simulink model "HybridShip_ModelE"  (R2026a)
settings: Solver=ode3  StopTime=7200  FixedStep=0.01
undefined symbols (not defined in the file): ADAPTER_FORCE_MODE, ADAPTER_FORCE_P1_KW, ADAPTER_FORCE_P2_KW, AI_Pred_Source, AI_TPeak_Source, ASSUMED_AI_DataValid, ASSUMED_Bat_Eff_Charge, ASSUMED_Bat_Eff_Discharge, ASSUMED_C_bus, ASSUMED_Drive_TimeConstant, ASSUMED_EMS_FF_Gain, ASSUMED_EMS_FF_Max_kW, ASSUMED_EMS_Manual_Pgen_kW, ASSUMED_EMS_SOC_Gain, ASSUMED_EMS_SOC_Ref, ASSUMED_eta_dcdc, ASSUMED_eta_rect, ASSUMED_Gen_TimeConstant, ASSUMED_K_droop, ASSUMED_Pred_Bound_kW, ASSUMED_SOC_ChgDerate_Start, ASSUMED_SOC_DisDerate_Start, ASSUMED_SOC_max, ASSUMED_SOC_min, ASSUMED_SpeedPI_Ki, ASSUMED_SpeedPI_Kp, ASSUMED_TFF_SOC_AdvancePct, ASSUMED_TFF_SOC_Thresh, ASSUMED_TFF_TauMargin, ASSUMED_V_floor, Bat_C1_LUT_F, Bat_eta_coul, Bat_I_limit_surrogate_A, Bat_OCV_LUT_V, Bat_P_conv_bus_max_kW, Bat_Q_nom_Ah, Bat_R0_chg_mult, Bat_R0_LUT_ohm, Bat_R1_LUT_ohm, Bat_SOC_init, Bat_SOC_LUT_nodes, Bat_V_max_V, Bat_V_min_V, BSFC_Breakpoints_kW, BSFC_Table_gkWh, CCS_Vdc_Steady_Band, CCS_Vdc_Transient_Band, DG_BSFC_gkWh, DG_BSFC_P_kW, DG_C_start_kg, DG_P_min_kW, DG_P_rated_kW, DG_ramp_kW_per_s, DG_t_starting_s, DG_t_sync_s, DG_tau_s, ECMS_dt_ctrl_s, ECMS_Grid_dP_kW, ECMS_Idle_Fuel_kgph, ECMS_K_S ... (+93)
libraries: simulink x8
(part 2 of 3)

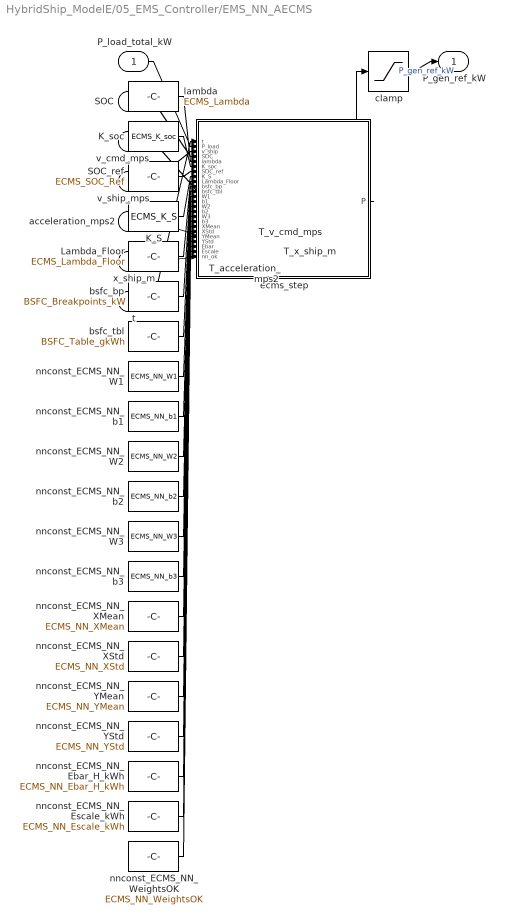
== system HybridShip_ModelE/05_EMS_Controller/EMS_NN_AECMS ==
  P_load_total_kW : Inport
  SOC : Inport  Port=2
  v_cmd_mps : Inport  Port=3
  v_ship_mps : Inport  Port=4
  acceleration_mps2 : Inport  Port=5
  x_ship_m : Inport  Port=6
  t : Inport  Port=7
  K_S : Constant  Value=ECMS_K_S
  K_soc : Constant  Value=ECMS_K_soc
  Lambda_Floor : Constant  Value=ECMS_Lambda_Floor
  SOC_ref : Constant  Value=ECMS_SOC_Ref
  T_acceleration_mps2 : Terminator
  T_v_cmd_mps : Terminator
  T_x_ship_m : Terminator
  bsfc_bp : Constant  Value=BSFC_Breakpoints_kW
  bsfc_tbl : Constant  Value=BSFC_Table_gkWh
  clamp : Saturate  UpperLimit=Gen_P_max  LowerLimit=0
  ecms_step : MATLAB Function  TreatAsAtomicUnit=on
  lambda : Constant  Value=ECMS_Lambda
  nnconst_ECMS_NN_Ebar_H_kWh : Constant  Value=ECMS_NN_Ebar_H_kWh
  nnconst_ECMS_NN_Escale_kWh : Constant  Value=ECMS_NN_Escale_kWh
  nnconst_ECMS_NN_W1 : Constant  Value=ECMS_NN_W1
  nnconst_ECMS_NN_W2 : Constant  Value=ECMS_NN_W2
  nnconst_ECMS_NN_W3 : Constant  Value=ECMS_NN_W3
  nnconst_ECMS_NN_WeightsOK : Constant  Value=ECMS_NN_WeightsOK
  nnconst_ECMS_NN_XMean : Constant  Value=ECMS_NN_XMean
  nnconst_ECMS_NN_XStd : Constant  Value=ECMS_NN_XStd
  nnconst_ECMS_NN_YMean : Constant  Value=ECMS_NN_YMean
  nnconst_ECMS_NN_YStd : Constant  Value=ECMS_NN_YStd
  nnconst_ECMS_NN_b1 : Constant  Value=ECMS_NN_b1
  nnconst_ECMS_NN_b2 : Constant  Value=ECMS_NN_b2
  nnconst_ECMS_NN_b3 : Constant  Value=ECMS_NN_b3
  P_gen_ref_kW : Outport
  wires:
  ? -> ?
  nnconst_ECMS_NN_W1/1 -> ecms_step/12(W1)
  nnconst_ECMS_NN_b1/1 -> ecms_step/13(b1)
  nnconst_ECMS_NN_W2/1 -> ecms_step/14(W2)
  nnconst_ECMS_NN_b2/1 -> ecms_step/15(b2)
  nnconst_ECMS_NN_W3/1 -> ecms_step/16(W3)
  nnconst_ECMS_NN_b3/1 -> ecms_step/17(b3)
  nnconst_ECMS_NN_XMean/1 -> ecms_step/18(XMean)
  nnconst_ECMS_NN_XStd/1 -> ecms_step/19(XStd)
  nnconst_ECMS_NN_YMean/1 -> ecms_step/20(YMean)
  nnconst_ECMS_NN_YStd/1 -> ecms_step/21(YStd)
  nnconst_ECMS_NN_Ebar_H_kWh/1 -> ecms_step/22(Ebar)
  nnconst_ECMS_NN_Escale_kWh/1 -> ecms_step/23(Escale)
  nnconst_ECMS_NN_WeightsOK/1 -> ecms_step/24(nn_ok)
  t/1 -> ecms_step/1(t)
  P_load_total_kW/1 -> ecms_step/2(P_load)
  v_ship_mps/1 -> ecms_step/3(v_ship)
  SOC/1 -> ecms_step/4(SOC)
  lambda/1 -> ecms_step/5(lambda)
  K_soc/1 -> ecms_step/6(K_soc)
  SOC_ref/1 -> ecms_step/7(SOC_ref)
  K_S/1 -> ecms_step/8(K_S)
  Lambda_Floor/1 -> ecms_step/9(Lambda_Floor)
  bsfc_bp/1 -> ecms_step/10(bsfc_bp)
  bsfc_tbl/1 -> ecms_step/11(bsfc_tbl)
  ecms_step/1(P) -> clamp/1
  clamp/1 -> P_gen_ref_kW/1  "P_gen_ref_kW"
  v_cmd_mps/1 -> T_v_cmd_mps/1
  acceleration_mps2/1 -> T_acceleration_mps2/1
  x_ship_m/1 -> T_x_ship_m/1

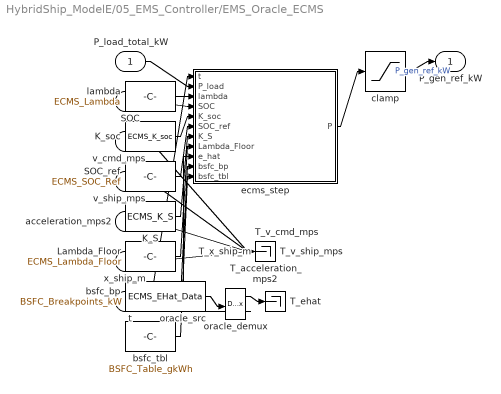
== system HybridShip_ModelE/05_EMS_Controller/EMS_Oracle_ECMS ==
  P_load_total_kW : Inport
  SOC : Inport  Port=2
  v_cmd_mps : Inport  Port=3
  v_ship_mps : Inport  Port=4
  acceleration_mps2 : Inport  Port=5
  x_ship_m : Inport  Port=6
  t : Inport  Port=7
  K_S : Constant  Value=ECMS_K_S
  K_soc : Constant  Value=ECMS_K_soc
  Lambda_Floor : Constant  Value=ECMS_Lambda_Floor
  SOC_ref : Constant  Value=ECMS_SOC_Ref
  T_acceleration_mps2 : Terminator
  T_ehat : Terminator
  T_v_cmd_mps : Terminator
  T_v_ship_mps : Terminator
  T_x_ship_m : Terminator
  bsfc_bp : Constant  Value=BSFC_Breakpoints_kW
  bsfc_tbl : Constant  Value=BSFC_Table_gkWh
  clamp : Saturate  UpperLimit=Gen_P_max  LowerLimit=0
  ecms_step : MATLAB Function  TreatAsAtomicUnit=on
  lambda : Constant  Value=ECMS_Lambda
  oracle_demux : Demux  Outputs=2
  oracle_src : FromWorkspace  VariableName=ECMS_EHat_Data  OutDataTypeStr=double  SampleTime=0.01  OutputAfterFinalValue=Holding final value
  P_gen_ref_kW : Outport
  wires:
  ? -> ?
  oracle_src/1 -> oracle_demux/1
  oracle_demux/2 -> ecms_step/9(e_hat)
  oracle_demux/1 -> T_ehat/1
  t/1 -> ecms_step/1(t)
  P_load_total_kW/1 -> ecms_step/2(P_load)
  lambda/1 -> ecms_step/3(lambda)
  SOC/1 -> ecms_step/4(SOC)
  K_soc/1 -> ecms_step/5(K_soc)
  SOC_ref/1 -> ecms_step/6(SOC_ref)
  K_S/1 -> ecms_step/7(K_S)
  Lambda_Floor/1 -> ecms_step/8(Lambda_Floor)
  bsfc_bp/1 -> ecms_step/10(bsfc_bp)
  bsfc_tbl/1 -> ecms_step/11(bsfc_tbl)
  ecms_step/1(P) -> clamp/1
  clamp/1 -> P_gen_ref_kW/1  "P_gen_ref_kW"
  v_cmd_mps/1 -> T_v_cmd_mps/1
  v_ship_mps/1 -> T_v_ship_mps/1
  acceleration_mps2/1 -> T_acceleration_mps2/1
  x_ship_m/1 -> T_x_ship_m/1

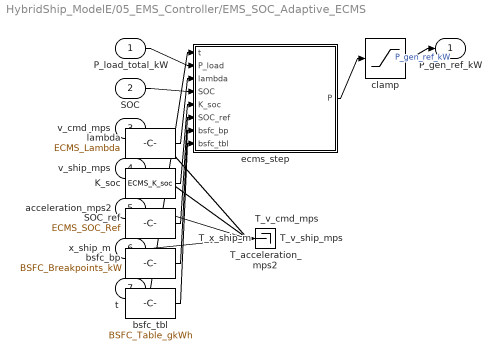
== system HybridShip_ModelE/05_EMS_Controller/EMS_SOC_Adaptive_ECMS ==
  P_load_total_kW : Inport
  SOC : Inport  Port=2
  v_cmd_mps : Inport  Port=3
  v_ship_mps : Inport  Port=4
  acceleration_mps2 : Inport  Port=5
  x_ship_m : Inport  Port=6
  t : Inport  Port=7
  K_soc : Constant  Value=ECMS_K_soc
  SOC_ref : Constant  Value=ECMS_SOC_Ref
  T_acceleration_mps2 : Terminator
  T_v_cmd_mps : Terminator
  T_v_ship_mps : Terminator
  T_x_ship_m : Terminator
  bsfc_bp : Constant  Value=BSFC_Breakpoints_kW
  bsfc_tbl : Constant  Value=BSFC_Table_gkWh
  clamp : Saturate  UpperLimit=Gen_P_max  LowerLimit=0
  ecms_step : MATLAB Function  TreatAsAtomicUnit=on
  lambda : Constant  Value=ECMS_Lambda
  P_gen_ref_kW : Outport
  wires:
  ? -> ?
  t/1 -> ecms_step/1(t)
  P_load_total_kW/1 -> ecms_step/2(P_load)
  lambda/1 -> ecms_step/3(lambda)
  SOC/1 -> ecms_step/4(SOC)
  K_soc/1 -> ecms_step/5(K_soc)
  SOC_ref/1 -> ecms_step/6(SOC_ref)
  bsfc_bp/1 -> ecms_step/7(bsfc_bp)
  bsfc_tbl/1 -> ecms_step/8(bsfc_tbl)
  ecms_step/1(P) -> clamp/1
  clamp/1 -> P_gen_ref_kW/1  "P_gen_ref_kW"
  v_cmd_mps/1 -> T_v_cmd_mps/1
  v_ship_mps/1 -> T_v_ship_mps/1
  acceleration_mps2/1 -> T_acceleration_mps2/1
  x_ship_m/1 -> T_x_ship_m/1

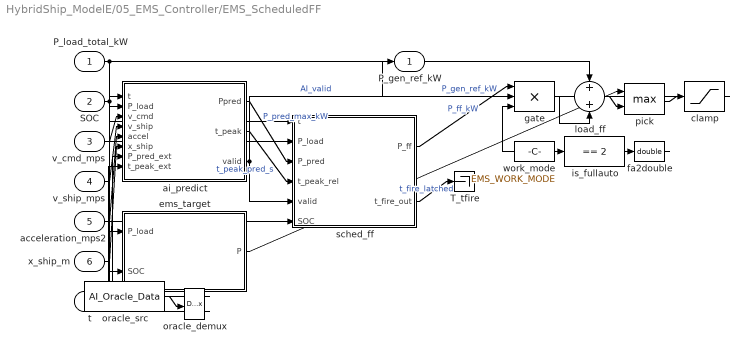
== system HybridShip_ModelE/05_EMS_Controller/EMS_ScheduledFF ==
  P_load_total_kW : Inport
  SOC : Inport  Port=2
  v_cmd_mps : Inport  Port=3
  v_ship_mps : Inport  Port=4
  acceleration_mps2 : Inport  Port=5
  x_ship_m : Inport  Port=6
  t : Inport  Port=7
  T_tfire : Terminator
  ai_predict : MATLAB Function  TreatAsAtomicUnit=on
  clamp : Saturate  UpperLimit=Gen_P_max  LowerLimit=0
  ems_target : MATLAB Function  TreatAsAtomicUnit=on
  fa2double : DataTypeConversion  OutDataTypeStr=double  SaturateOnIntegerOverflow=off  RndMeth=Floor
  gate : Product  Inputs=***
  is_fullauto : simulink/Logic and Bit Operations/Compare To Constant  relop===  const=2  OutDataTypeStr=boolean
  load_ff : Sum
  oracle_demux : Demux  Outputs=2
  oracle_src : FromWorkspace  VariableName=AI_Oracle_Data  OutDataTypeStr=double  SampleTime=0.01  OutputAfterFinalValue=Holding final value
  pick : MinMax  Function=max  Inputs=2
  sched_ff : MATLAB Function  TreatAsAtomicUnit=on
  work_mode : Constant  Value=EMS_WORK_MODE
  P_gen_ref_kW : Outport
  wires:
  ? -> ?
  oracle_src/1 -> oracle_demux/1
  oracle_demux/1 -> ai_predict/7(P_pred_ext)
  oracle_demux/2 -> ai_predict/8(t_peak_ext)
  t/1 -> ai_predict/1(t), sched_ff/1(t)
  P_load_total_kW/1 -> ai_predict/2(P_load), ems_target/1(P_load), sched_ff/2(P_load), load_ff/1
  v_cmd_mps/1 -> ai_predict/3(v_cmd)
  v_ship_mps/1 -> ai_predict/4(v_ship)
  acceleration_mps2/1 -> ai_predict/5(accel)
  x_ship_m/1 -> ai_predict/6(x_ship)
  SOC/1 -> ems_target/2(SOC), sched_ff/6(SOC)
  ai_predict/1(Ppred) -> sched_ff/3(P_pred)  "P_pred_max_kW"
  ai_predict/2(t_peak) -> sched_ff/4(t_peak_rel)  "t_peak_pred_s"
  ai_predict/3(valid) -> sched_ff/5(valid), gate/2  "AI_valid"
  sched_ff/1(P_ff) -> gate/1  "P_ff_kW"
  sched_ff/2(t_fire_out) -> T_tfire/1  "t_fire_latched"
  work_mode/1 -> is_fullauto/1
  is_fullauto/1 -> fa2double/1
  fa2double/1 -> gate/3
  gate/1 -> load_ff/2
  ems_target/1(P) -> pick/1
  load_ff/1 -> pick/2
  pick/1 -> clamp/1
  clamp/1 -> P_gen_ref_kW/1  "P_gen_ref_kW"

== matlab function HybridShip_ModelE/03_Propulsion_Plant/Wake_vs_HT ==
  data: HT_ratio input; w output; Wake_w_deep parameter; Wake_HT_nodes parameter; Wake_w_Zhang parameter; Wake_HT_ref parameter; Wake_w_ref parameter
function w = WakeVsHT(HT_ratio, Wake_w_deep, Wake_HT_nodes, Wake_w_Zhang, Wake_HT_ref, Wake_w_ref)
% Wake_vs_HT —— 伴流分数 w(H/T) = w_deep + Δw_Zhang(H/T)（OQ-4/D-3，design §4.2，T-005）
% 【transferred literature surrogate 声明】Δw 取自 Zhang 2023 双桨表（标定族 C_B=0.86 与
% 本船 C_B=0.60 不同），只借相对变化量；不得表述为本船验证伴流场。
% 深水锚 w_deep 由 Harvald/Molland 回归独立确定（D-3），非 Zhang 绝对值。
% 域处理（与船体模块 clamp 语义一致）：
%   H/T > Wake_HT_ref(2.7)      -> Δw = 0（深水渐近，显式分支，不依赖插值未定义行为）
%   H/T < min(Wake_HT_nodes)    -> clamp 到首节点 1.2（与船体模块 clamp 一致）
%   其间 linear 插值（防 overshoot），查询域 clamp [1.2, Wake_HT_ref]
if HT_ratio > Wake_HT_ref
    w = Wake_w_deep;   % 深水渐近：Δw = 0
else
    wHT = min(max(HT_ratio, min(Wake_HT_nodes)), Wake_HT_ref);
    w = Wake_w_deep + (interp1(Wake_HT_nodes, Wake_w_Zhang, wHT, 'linear') - Wake_w_ref);
end
end

== matlab function HybridShip_ModelE/03_Propulsion_Plant/Ship_Hull_Dynamics_E ==
  data: V_ship input; dVdt output; F_prop_eff input; V_current input; F_env input; resistance_multiplier input; water_depth_m input; R_total_N output; R_shallow_N output; HT_ratio output; domain_warning output; Hull_K_R parameter; Ship_Mass parameter; Hull_Lpp_m parameter; Hull_T_m parameter; nu_water parameter; Hull_k_form parameter; Shallow_c1 parameter; Shallow_c2 parameter; Shallow_c3 parameter; Shallow_HT_deep_limit parameter; Shallow_HT_min_valid parameter
function [dVdt, R_total_N, R_shallow_N, HT_ratio, domain_warning] = ShipHullDynamicsE(...
    V_ship, F_prop_eff, V_current, F_env, resistance_multiplier, water_depth_m, ...
    Hull_K_R, Ship_Mass, Hull_Lpp_m, Hull_T_m, nu_water, Hull_k_form, ...
Shallow_c1, Shallow_c2, Shallow_c3, Shallow_HT_deep_limit, Shallow_HT_min_valid)
% Ship_Hull_Dynamics_E —— 船体纵向动力学 + 浅水相对增量阻力（design §4.1，FR-412~415，T-004）
% 相对增量法：文献公式只计算无量纲浅水增量 Δr(H/T, Re)，绝对阻力水平由 Hull_K_R 锚定
% 域处理（FR-415，禁静默外推）：
%   H/T > Shallow_HT_deep_limit(3.0) -> Δr = 0（深水渐近）
%   H/T < Shallow_HT_min_valid(1.2)  -> clamp 到 1.2 计算 + domain_warning = 1
%   其间正常计算，domain_warning = 0
% 数值稳健（NFR-411）：零速跳过浅水项（Re=0 -> log10 发散 -> 0/0 NaN），Re 下限保护 1e3，
%   全程无 NaN/Inf
% 已知局限（证据链登记）：c1/c2/c3 标定族 C_B=0.86 与本船 0.60 型差外推；
%   未含浅水兴波临界区（Fr_h->1）分量，由 H/T>=1.2 域限 + C 包 UKC 限速规避
V_rel = V_ship - V_current;
HT_ratio = water_depth_m / Hull_T_m;
domain_warning = 0;
HT_eff = HT_ratio;
shallow_active = true;
if HT_ratio > Shallow_HT_deep_limit
    shallow_active = false;   % 深水渐近：Δr = 0
elseif HT_ratio < Shallow_HT_min_valid
    HT_eff = Shallow_HT_min_valid;   % clamp 到下界（禁静默外推）
    domain_warning = 1;              % MODEL_DOMAIN_WARNING（NFR-411）
end
if abs(V_rel) < eps
    R_total_N = 0;
    R_shallow_N = 0;
    dVdt = (F_prop_eff + F_env) / Ship_Mass;
    return;
end
R_deep = resistance_multiplier * Hull_K_R * V_rel * abs(V_rel);
R_shallow_N = 0;
if shallow_active
    Re = max(abs(V_rel) * Hull_Lpp_m / nu_water, 1e3);   % Re 下限保护（NFR-411）
    Lr = log10(Re);
    C_F = 0.075 / (Lr - 2)^2;                            % ITTC-57 摩擦阻力系数
    C_Fstar = 0.08468 / (Lr - 1.631)^2 * ...
        (1 + Shallow_c1 / (Lr + Shallow_c2) * HT_eff^Shallow_c3);   % Zhang/Rhine86 [1][3]
    deltak = 0.644 * HT_eff^(-1.72);   % Millward[4]/Zhang[1]：系数 0.644 与指数 -1.72 字面量
    deltar = (1 + Hull_k_form + deltak) * C_Fstar / ((1 + Hull_k_form) * C_F) - 1;
    R_shallow_N = R_deep * deltar;   % Δr 为相对增量：R_shallow 是浅水附加量（FR-413）
end
R_total_N = R_deep + R_shallow_N;   % = R_deep*(1+Δr)
dVdt = (F_prop_eff - R_total_N + F_env) / Ship_Mass;
end

== matlab function HybridShip_ModelE/05_EMS_Controller/EMS_Baseline/ems_target ==
  data: P_load input; P output; SOC input; EMS_WORK_MODE parameter; ASSUMED_EMS_Manual_Pgen_kW parameter; ASSUMED_EMS_SOC_Gain parameter; ASSUMED_EMS_SOC_Ref parameter
function P = ems_target(P_load, SOC, EMS_WORK_MODE, ASSUMED_EMS_Manual_Pgen_kW, ASSUMED_EMS_SOC_Gain, ASSUMED_EMS_SOC_Ref)
% EMS 三模式：0=手动(定功率只监测) 1=半自动(负荷跟随+SOC修正) 2=全自动
if EMS_WORK_MODE == 0
    P = ASSUMED_EMS_Manual_Pgen_kW;
else
    P = P_load + ASSUMED_EMS_SOC_Gain * (ASSUMED_EMS_SOC_Ref - SOC);
end
end

== matlab function HybridShip_ModelE/05_EMS_Controller/EMS_AI_Enhanced/ai_predict ==
  settings: updateMethod=DISCRETE  sampleTime=0.01
  data: t input; Ppred output; P_load input; v_cmd input; v_ship input; accel input; x_ship input; P_pred_ext input; t_peak_ext input; t_peak output; valid output; AI_Pred_Source parameter; AI_TPeak_Source parameter; ASSUMED_AI_DataValid parameter; ASSUMED_Pred_Bound_kW parameter; MLP_WeightsLoaded parameter; MLP_W1 parameter size=[110 64]; MLP_b1 parameter size=[1 64]; MLP_W2 parameter size=[64 32]; MLP_b2 parameter size=[1 32]; MLP_W3 parameter size=[32 1]; MLP_b3 parameter size=[1 1]; MLP_FeatMean parameter size=[1 5]; MLP_FeatStd parameter size=[1 5]; MLP_YMean parameter size=[1 1]; MLP_YStd parameter size=[1 1]
function [Ppred, t_peak, valid] = ai_predict(t, P_load, v_cmd, v_ship, accel, x_ship, P_pred_ext, t_peak_ext, AI_Pred_Source, AI_TPeak_Source, ASSUMED_AI_DataValid, ASSUMED_Pred_Bound_kW, MLP_WeightsLoaded, MLP_W1, MLP_b1, MLP_W2, MLP_b2, MLP_W3, MLP_b3, MLP_FeatMean, MLP_FeatStd, MLP_YMean, MLP_YStd)
% AI 预测接口：输出预测峰值功率 P_pred_max_kW、到达时间 t_peak_pred_s 与有效性 AI_valid
% AI_Pred_Source: 0=Disabled/Persistence, 1=FromWorkspace, 2=External(STM32N6 预留), 3=EmbeddedML(环内 MLP 推理)
% AI_TPeak_Source: 0=按 AI_Pred_Source 语义取 t_peak; 1=强制取 t_peak_ext(真值, E3 用)
% P_pred_ext/t_peak_ext: 外部预测信号（来自变体内 From Workspace 块读 AI_Oracle_Data N×3）
% 注意：EMChart 局部函数不可见图级参数，MLP 推理全部内联于主函数（2026-08 调试结论）
persistent hist lastT
if isempty(hist)
    hist = repmat([P_load, v_cmd, v_ship, accel, x_ship], 22, 1);
    lastT = t - 1;
end
if t - lastT >= 1 - 1e-9
    hist = [hist(2:end, :); P_load, v_cmd, v_ship, accel, x_ship];
    lastT = t;
end
t_peak = 0;
if AI_Pred_Source == 0
    Ppred = P_load; valid = 1;
elseif AI_Pred_Source == 3
    if MLP_WeightsLoaded < 0.5
        Ppred = P_load; valid = 0;
        return;
    end
    x = reshape(hist.', 1, []);
    mu = repmat(MLP_FeatMean, 1, 22);
    sd = repmat(MLP_FeatStd, 1, 22);
    xn = (x - mu) ./ sd;
    h1 = max(xn * MLP_W1 + MLP_b1, 0);
    h2 = max(h1 * MLP_W2 + MLP_b2, 0);
    yn = h2 * MLP_W3 + MLP_b3;
    delta = max(yn * MLP_YStd + MLP_YMean, 0);
    Ppred = P_load + delta;
    ok = all(isfinite([Ppred, P_load, v_cmd, v_ship, accel, x_ship]));
    ok = ok && Ppred >= 0 && Ppred <= ASSUMED_Pred_Bound_kW;
    valid = double(ok);
    Ppred = min(max(Ppred, 0), ASSUMED_Pred_Bound_kW);
else
    % AI_Pred_Source == 1 | 2：外部预测信号（From Workspace / STM32N6 预留）
    if ASSUMED_AI_DataValid
        Ppred = P_pred_ext;
        t_peak = t_peak_ext;
        ok = all(isfinite([Ppred, t_peak, P_load, v_cmd, v_ship, accel, x_ship]));
        ok = ok && Ppred >= 0 && Ppred <= ASSUMED_Pred_Bound_kW;
        ok = ok && t_peak >= 0 && t_peak <= 60;
        valid = double(ok);
        Ppred = min(max(Ppred, 0), ASSUMED_Pred_Bound_kW);
        t_peak = min(max(t_peak, 0), 60);
    else
        Ppred = P_load; valid = 0;
        return;
    end
end
if AI_TPeak_Source == 1 && AI_Pred_Source ~= 0
    % E3：MLP 幅值 + oracle t_peak 真值覆盖（防御性裁剪）
    if isfinite(t_peak_ext)
        t_peak = min(max(t_peak_ext, 0), 60);
    else
        t_peak = 0;
    end
end
end

== matlab function HybridShip_ModelE/05_EMS_Controller/EMS_AI_Enhanced/ems_target ==
  data: P_load input; P output; SOC input; EMS_WORK_MODE parameter; ASSUMED_EMS_Manual_Pgen_kW parameter; ASSUMED_EMS_SOC_Gain parameter; ASSUMED_EMS_SOC_Ref parameter
function P = ems_target(P_load, SOC, EMS_WORK_MODE, ASSUMED_EMS_Manual_Pgen_kW, ASSUMED_EMS_SOC_Gain, ASSUMED_EMS_SOC_Ref)
% EMS 三模式：0=手动(定功率只监测) 1=半自动(负荷跟随+SOC修正) 2=全自动
if EMS_WORK_MODE == 0
    P = ASSUMED_EMS_Manual_Pgen_kW;
else
    P = P_load + ASSUMED_EMS_SOC_Gain * (ASSUMED_EMS_SOC_Ref - SOC);
end
end

== matlab function HybridShip_ModelE/05_EMS_Controller/EMS_ScheduledFF/ai_predict ==
  settings: updateMethod=DISCRETE  sampleTime=0.01
  data: t input; Ppred output; P_load input; v_cmd input; v_ship input; accel input; x_ship input; P_pred_ext input; t_peak_ext input; t_peak output; valid output; AI_Pred_Source parameter; AI_TPeak_Source parameter; ASSUMED_AI_DataValid parameter; ASSUMED_Pred_Bound_kW parameter; MLP_WeightsLoaded parameter; MLP_W1 parameter size=[110 64]; MLP_b1 parameter size=[1 64]; MLP_W2 parameter size=[64 32]; MLP_b2 parameter size=[1 32]; MLP_W3 parameter size=[32 1]; MLP_b3 parameter size=[1 1]; MLP_FeatMean parameter size=[1 5]; MLP_FeatStd parameter size=[1 5]; MLP_YMean parameter size=[1 1]; MLP_YStd parameter size=[1 1]
function [Ppred, t_peak, valid] = ai_predict(t, P_load, v_cmd, v_ship, accel, x_ship, P_pred_ext, t_peak_ext, AI_Pred_Source, AI_TPeak_Source, ASSUMED_AI_DataValid, ASSUMED_Pred_Bound_kW, MLP_WeightsLoaded, MLP_W1, MLP_b1, MLP_W2, MLP_b2, MLP_W3, MLP_b3, MLP_FeatMean, MLP_FeatStd, MLP_YMean, MLP_YStd)
% AI 预测接口：输出预测峰值功率 P_pred_max_kW、到达时间 t_peak_pred_s 与有效性 AI_valid
% AI_Pred_Source: 0=Disabled/Persistence, 1=FromWorkspace, 2=External(STM32N6 预留), 3=EmbeddedML(环内 MLP 推理)
% AI_TPeak_Source: 0=按 AI_Pred_Source 语义取 t_peak; 1=强制取 t_peak_ext(真值, E3 用)
% P_pred_ext/t_peak_ext: 外部预测信号（来自变体内 From Workspace 块读 AI_Oracle_Data N×3）
% 注意：EMChart 局部函数不可见图级参数，MLP 推理全部内联于主函数（2026-08 调试结论）
persistent hist lastT
if isempty(hist)
    hist = repmat([P_load, v_cmd, v_ship, accel, x_ship], 22, 1);
    lastT = t - 1;
end
if t - lastT >= 1 - 1e-9
    hist = [hist(2:end, :); P_load, v_cmd, v_ship, accel, x_ship];
    lastT = t;
end
t_peak = 0;
if AI_Pred_Source == 0
    Ppred = P_load; valid = 1;
elseif AI_Pred_Source == 3
    if MLP_WeightsLoaded < 0.5
        Ppred = P_load; valid = 0;
        return;
    end
    x = reshape(hist.', 1, []);
    mu = repmat(MLP_FeatMean, 1, 22);
    sd = repmat(MLP_FeatStd, 1, 22);
    xn = (x - mu) ./ sd;
    h1 = max(xn * MLP_W1 + MLP_b1, 0);
    h2 = max(h1 * MLP_W2 + MLP_b2, 0);
    yn = h2 * MLP_W3 + MLP_b3;
    delta = max(yn * MLP_YStd + MLP_YMean, 0);
    Ppred = P_load + delta;
    ok = all(isfinite([Ppred, P_load, v_cmd, v_ship, accel, x_ship]));
    ok = ok && Ppred >= 0 && Ppred <= ASSUMED_Pred_Bound_kW;
    valid = double(ok);
    Ppred = min(max(Ppred, 0), ASSUMED_Pred_Bound_kW);
else
    % AI_Pred_Source == 1 | 2：外部预测信号（From Workspace / STM32N6 预留）
    if ASSUMED_AI_DataValid
        Ppred = P_pred_ext;
        t_peak = t_peak_ext;
        ok = all(isfinite([Ppred, t_peak, P_load, v_cmd, v_ship, accel, x_ship]));
        ok = ok && Ppred >= 0 && Ppred <= ASSUMED_Pred_Bound_kW;
        ok = ok && t_peak >= 0 && t_peak <= 60;
        valid = double(ok);
        Ppred = min(max(Ppred, 0), ASSUMED_Pred_Bound_kW);
        t_peak = min(max(t_peak, 0), 60);
    else
        Ppred = P_load; valid = 0;
        return;
    end
end
if AI_TPeak_Source == 1 && AI_Pred_Source ~= 0
    % E3：MLP 幅值 + oracle t_peak 真值覆盖（防御性裁剪）
    if isfinite(t_peak_ext)
        t_peak = min(max(t_peak_ext, 0), 60);
    else
        t_peak = 0;
    end
end
end

== matlab function HybridShip_ModelE/05_EMS_Controller/EMS_ScheduledFF/ems_target ==
  data: P_load input; P output; SOC input; EMS_WORK_MODE parameter; ASSUMED_EMS_Manual_Pgen_kW parameter; ASSUMED_EMS_SOC_Gain parameter; ASSUMED_EMS_SOC_Ref parameter
function P = ems_target(P_load, SOC, EMS_WORK_MODE, ASSUMED_EMS_Manual_Pgen_kW, ASSUMED_EMS_SOC_Gain, ASSUMED_EMS_SOC_Ref)
% EMS 三模式：0=手动(定功率只监测) 1=半自动(负荷跟随+SOC修正) 2=全自动
if EMS_WORK_MODE == 0
    P = ASSUMED_EMS_Manual_Pgen_kW;
else
    P = P_load + ASSUMED_EMS_SOC_Gain * (ASSUMED_EMS_SOC_Ref - SOC);
end
end

== matlab function HybridShip_ModelE/05_EMS_Controller/EMS_ScheduledFF/sched_ff ==
  settings: updateMethod=DISCRETE  sampleTime=0.01
  data: t input; P_ff output; P_load input; P_pred input; t_peak_rel input; valid input; SOC input; t_fire_out output; Gen_Ramp_Up parameter; ASSUMED_TFF_TauMargin parameter; ASSUMED_TFF_SOC_Thresh parameter; ASSUMED_TFF_SOC_AdvancePct parameter; ASSUMED_EMS_FF_Gain parameter; ASSUMED_EMS_FF_Max_kW parameter; ASSUMED_Gen_TimeConstant parameter
function [P_ff, t_fire_out] = sched_ff(t, P_load, P_pred, t_peak_rel, valid, SOC, Gen_Ramp_Up, ASSUMED_TFF_TauMargin, ASSUMED_TFF_SOC_Thresh, ASSUMED_TFF_SOC_AdvancePct, ASSUMED_EMS_FF_Gain, ASSUMED_EMS_FF_Max_kW, ASSUMED_Gen_TimeConstant)
% 定时前馈核心控制律（T-004）：
%   输入: t(当前绝对时间), P_load, P_pred(预测峰值), t_peak_rel(相对秒数), valid, SOC
%   输出: P_ff(前馈功率), t_fire_out(触发时刻,无事件时 -1)
%   刷新: 每 1 Hz 与 ai_predict 刷新对齐（t-lastT>=1）；每 0.01 s 步输出
persistent ev_active ev_immediate ev_tFire ev_tPeakAbs ev_dP lastT
if isempty(ev_active)
    ev_active = false; ev_immediate = false;
    ev_tFire = 0; ev_tPeakAbs = 0; ev_dP = 0;
    lastT = t - 1;
end
if t - lastT >= 1 - 1e-9
    lastT = t;
    dP = min(max(P_pred - P_load, 0) * ASSUMED_EMS_FF_Gain, ASSUMED_EMS_FF_Max_kW);
    if dP <= 0 || valid < 0.5
        ev_active = false; ev_immediate = false;
        ev_tFire = 0; ev_tPeakAbs = 0; ev_dP = 0;
    else
        T_ramp = dP / Gen_Ramp_Up + ASSUMED_TFF_TauMargin;
        if SOC < ASSUMED_TFF_SOC_Thresh
            T_ramp = T_ramp * (1 + ASSUMED_TFF_SOC_AdvancePct);
        end
        if t_peak_rel <= T_ramp
            % 来不及 → 立即模式（退化 C1）
            ev_active = true; ev_immediate = true;
            ev_dP = dP; ev_tFire = t; ev_tPeakAbs = t + t_peak_rel;
        elseif ev_active && ~ev_immediate && t < ev_tFire
            % 等待期：跟随最新预测重排
            ev_dP = dP; ev_tFire = t + t_peak_rel - T_ramp; ev_tPeakAbs = t + t_peak_rel;
        elseif ev_active && t >= ev_tFire
            % 锁存期：ΔP 只增不减，峰值时间只延不缩
            ev_dP = max(ev_dP, dP); ev_tPeakAbs = max(ev_tPeakAbs, t + t_peak_rel);
        else
            % 新事件
            ev_active = true; ev_immediate = false;
            ev_dP = dP; ev_tFire = t + t_peak_rel - T_ramp; ev_tPeakAbs = t + t_peak_rel;
        end
    end
end
% 每个 0.01 s 步输出
P_ff = 0; t_fire_out = -1;
if ev_active
    if t > ev_tPeakAbs + ASSUMED_Gen_TimeConstant
        % 峰值过后释放
        ev_active = false; ev_immediate = false;
        ev_tFire = 0; ev_tPeakAbs = 0; ev_dP = 0;
    else
        t_fire_out = ev_tFire;
        if ev_immediate || t >= ev_tFire
            P_ff = ev_dP;
        end
    end
end
end

== matlab function HybridShip_ModelE/05_EMS_Controller/EMS_Fixed_ECMS/ecms_step ==
  settings: updateMethod=DISCRETE  sampleTime=0.01
  data: t input; P output; P_load input; lambda input; SOC input; bsfc_bp input; bsfc_tbl input; ASSUMED_eta_rect parameter; ASSUMED_eta_dcdc parameter; ASSUMED_Bat_Eff_Discharge parameter; ASSUMED_Bat_Eff_Charge parameter; Gen_P_max parameter; ECMS_SOC_Discharge_Max parameter; ECMS_SOC_Charge_Min parameter; ECMS_Idle_Fuel_kgph parameter; ECMS_Grid_dP_kW parameter; ECMS_dt_ctrl_s parameter; Pgen_init parameter
function P = ecms_fixed(t, P_load, lambda, SOC, bsfc_bp, bsfc_tbl, ASSUMED_eta_rect, ASSUMED_eta_dcdc, ASSUMED_Bat_Eff_Discharge, ASSUMED_Bat_Eff_Charge, Gen_P_max, ECMS_SOC_Discharge_Max, ECMS_SOC_Charge_Min, ECMS_Idle_Fuel_kgph, ECMS_Grid_dP_kW, ECMS_dt_ctrl_s, Pgen_init)
% Fixed ECMS（law=4，T-103）：单步网格穷举（design §3.1）
% 与离线参考 +ecms2/ecms_law.m 逐位一致（+ecms2/test_ecms_law.m 单测5 容差0锁定）
% 控制周期 ECMS_dt_ctrl_s=1 s：内部持久门控，更新间隔内保持输出
persistent lastT Pheld
if isempty(lastT)
    lastT = -1e9;
    Pheld = Pgen_init;
end
P = Pheld;
if t - lastT < ECMS_dt_ctrl_s - 1e-9
    return;
end
lastT = t;
% 可行集 = {0（怠速）} ∪ [0:ECMS_Grid_dP_kW:Gen_P_max]（P_min=0 口径）
N = floor(Gen_P_max / ECMS_Grid_dP_kW) + 1;
Pbest = 0;
Jbest = inf;
nb = numel(bsfc_bp);
for i = 1:N
    Pg = (i - 1) * ECMS_Grid_dP_kW;
    Pbat = P_load - ASSUMED_eta_rect * Pg;
    % SOC 硬约束（优先于 λ）：禁放电 -> 取满足需求的最小可行值
    if SOC <= ECMS_SOC_Discharge_Max
        if Pbat > 1e-9
            continue;
        end
        Pbest = Pg;
        break;
    end
    % SOC 硬约束：禁充电（排除充电网格点）
    if SOC >= ECMS_SOC_Charge_Min && Pbat < 0
        continue;
    end
    % ṁ_f：怠速（Pg=0）用怠速流量，否则 Pg·bsfc(Pg)/3.6e6
    if Pg < 1e-9
        mf = ECMS_Idle_Fuel_kgph / 3600;
    else
        bsfc = bsfc_tbl(1);
        if Pg >= bsfc_bp(nb)
            bsfc = bsfc_tbl(nb);
        elseif Pg > bsfc_bp(1)
            ii = 1;
            while ii < nb - 1 && bsfc_bp(ii + 1) < Pg
                ii = ii + 1;
            end
            w = (Pg - bsfc_bp(ii)) / (bsfc_bp(ii + 1) - bsfc_bp(ii));
            bsfc = bsfc_tbl(ii) + w * (bsfc_tbl(ii + 1) - bsfc_tbl(ii));
        end
        mf = Pg * bsfc / 3.6e6;
    end
    % ṁ_bat,eq：放电正代价，充电负收益（design §3.1 效率链）
    if Pbat > 0
        mbe = Pbat / (ASSUMED_eta_dcdc * ASSUMED_Bat_Eff_Discharge) / 3600;
    else
        mbe = Pbat * (ASSUMED_eta_dcdc * ASSUMED_Bat_Eff_Charge) / 3600;
    end
    J = mf + lambda * mbe;
    if J < Jbest
        Jbest = J;
        Pbest = Pg;
    end
end
% 禁放电且需求 > η_rect·P_max（无网格点可满足）-> 尽力最大
if SOC <= ECMS_SOC_Discharge_Max && Pbest < 1e-9 && P_load > ASSUMED_eta_rect * Gen_P_max
    Pbest = Gen_P_max;
end
P = Pbest;
Pheld = Pbest;
end

== matlab function HybridShip_ModelE/05_EMS_Controller/EMS_SOC_Adaptive_ECMS/ecms_step ==
  settings: updateMethod=DISCRETE  sampleTime=0.01
  data: t input; P output; P_load input; lambda input; SOC input; K_soc input; SOC_ref input; bsfc_bp input; bsfc_tbl input; ASSUMED_eta_rect parameter; ASSUMED_eta_dcdc parameter; ASSUMED_Bat_Eff_Discharge parameter; ASSUMED_Bat_Eff_Charge parameter; Gen_P_max parameter; ECMS_SOC_Discharge_Max parameter; ECMS_SOC_Charge_Min parameter; ECMS_Idle_Fuel_kgph parameter; ECMS_Grid_dP_kW parameter; ECMS_dt_ctrl_s parameter; Pgen_init parameter
function P = ecms_adaptive(t, P_load, lambda, SOC, K_soc, SOC_ref, bsfc_bp, bsfc_tbl, ASSUMED_eta_rect, ASSUMED_eta_dcdc, ASSUMED_Bat_Eff_Discharge, ASSUMED_Bat_Eff_Charge, Gen_P_max, ECMS_SOC_Discharge_Max, ECMS_SOC_Charge_Min, ECMS_Idle_Fuel_kgph, ECMS_Grid_dP_kW, ECMS_dt_ctrl_s, Pgen_init)
% SOC-Adaptive ECMS（law=5，T-105）：λ(t) = λ₀ + K_soc·(SOC_ref − SOC)（design §3.2）
% 与离线参考 +ecms2/ecms_law.m（law=5）逐位一致（+ecms2/test_ecms_law.m 单测7 容差0锁定）
% 控制周期 ECMS_dt_ctrl_s=1 s：内部持久门控，更新间隔内保持输出
persistent lastT Pheld
if isempty(lastT)
    lastT = -1e9;
    Pheld = Pgen_init;
end
P = Pheld;
if t - lastT < ECMS_dt_ctrl_s - 1e-9
    return;
end
lastT = t;
% 自适应 λ：SOC 高于 SOC_ref -> λ 下降（电池更便宜）；低于 -> λ 上升
lam = lambda + K_soc * (SOC_ref - SOC);
% 可行集 = {0（怠速）} ∪ [0:ECMS_Grid_dP_kW:Gen_P_max]（P_min=0 口径）
N = floor(Gen_P_max / ECMS_Grid_dP_kW) + 1;
Pbest = 0;
Jbest = inf;
nb = numel(bsfc_bp);
for i = 1:N
    Pg = (i - 1) * ECMS_Grid_dP_kW;
    Pbat = P_load - ASSUMED_eta_rect * Pg;
    % SOC 硬约束（优先于 λ）：禁放电 -> 取满足需求的最小可行值
    if SOC <= ECMS_SOC_Discharge_Max
        if Pbat > 1e-9
            continue;
        end
        Pbest = Pg;
        break;
    end
    % SOC 硬约束：禁充电（排除充电网格点）
    if SOC >= ECMS_SOC_Charge_Min && Pbat < 0
        continue;
    end
    % ṁ_f：怠速（Pg=0）用怠速流量，否则 Pg·bsfc(Pg)/3.6e6
    if Pg < 1e-9
        mf = ECMS_Idle_Fuel_kgph / 3600;
    else
        bsfc = bsfc_tbl(1);
        if Pg >= bsfc_bp(nb)
            bsfc = bsfc_tbl(nb);
        elseif Pg > bsfc_bp(1)
            ii = 1;
            while ii < nb - 1 && bsfc_bp(ii + 1) < Pg
                ii = ii + 1;
            end
            w = (Pg - bsfc_bp(ii)) / (bsfc_bp(ii + 1) - bsfc_bp(ii));
            bsfc = bsfc_tbl(ii) + w * (bsfc_tbl(ii + 1) - bsfc_tbl(ii));
        end
        mf = Pg * bsfc / 3.6e6;
    end
    % ṁ_bat,eq：放电正代价，充电负收益（design §3.1 效率链）
    if Pbat > 0
        mbe = Pbat / (ASSUMED_eta_dcdc * ASSUMED_Bat_Eff_Discharge) / 3600;
    else
        mbe = Pbat * (ASSUMED_eta_dcdc * ASSUMED_Bat_Eff_Charge) / 3600;
    end
    J = mf + lam * mbe;
    if J < Jbest
        Jbest = J;
        Pbest = Pg;
    end
end
% 禁放电且需求 > η_rect·P_max（无网格点可满足）-> 尽力最大
if SOC <= ECMS_SOC_Discharge_Max && Pbest < 1e-9 && P_load > ASSUMED_eta_rect * Gen_P_max
    Pbest = Gen_P_max;
end
P = Pbest;
Pheld = Pbest;
end

== matlab function HybridShip_ModelE/05_EMS_Controller/EMS_Oracle_ECMS/ecms_step ==
  settings: updateMethod=DISCRETE  sampleTime=0.01
  data: t input; P output; P_load input; lambda input; SOC input; K_soc input; SOC_ref input; K_S input; Lambda_Floor input; e_hat input; bsfc_bp input; bsfc_tbl input; ASSUMED_eta_rect parameter; ASSUMED_eta_dcdc parameter; ASSUMED_Bat_Eff_Discharge parameter; ASSUMED_Bat_Eff_Charge parameter; Gen_P_max parameter; ECMS_SOC_Discharge_Max parameter; ECMS_SOC_Charge_Min parameter; ECMS_Idle_Fuel_kgph parameter; ECMS_Grid_dP_kW parameter; ECMS_dt_ctrl_s parameter; Pgen_init parameter
function P = ecms_oracle(t, P_load, lambda, SOC, K_soc, SOC_ref, K_S, Lambda_Floor, e_hat, bsfc_bp, bsfc_tbl, ASSUMED_eta_rect, ASSUMED_eta_dcdc, ASSUMED_Bat_Eff_Discharge, ASSUMED_Bat_Eff_Charge, Gen_P_max, ECMS_SOC_Discharge_Max, ECMS_SOC_Charge_Min, ECMS_Idle_Fuel_kgph, ECMS_Grid_dP_kW, ECMS_dt_ctrl_s, Pgen_init)
% Oracle Predictive A-ECMS（law=6，T-106，design v1.1）：
%   SOC_ref_eff = SOC_ref + K_S*e_hat；λ_eff = λ₀ + K_soc*(SOC_ref_eff − SOC)；
%   λ_eff = max(λ_eff, Lambda_Floor)（下限钳位，防发电塌缩支路）。
% 预测改走 SOC_ref 通道（v2；v1 直接加法 K_E·ê 已在 S20 证伪，见 kE_calibration.json）。
% 与离线参考 +ecms2/ecms_law.m（law=6）逐位一致（+ecms2/test_ecms_law.m 单测9 容差0锁定）。
% 控制周期 ECMS_dt_ctrl_s=1 s。红线（E5）：ê_future 为 oracle 离线预计算
% （ECMS_EHat_Data，真实未来需求），非实时可实现——law=6 仅用于上界/增量验证。
persistent lastT Pheld
if isempty(lastT)
    lastT = -1e9;
    Pheld = Pgen_init;
end
P = Pheld;
if t - lastT < ECMS_dt_ctrl_s - 1e-9
    return;
end
lastT = t;
% 自适应 λ（v2）：前瞻 ê>0 -> SOC_ref 升 -> λ 升（保电）；ê<0 -> SOC_ref 降；
% 下限钳位仅当 oracle 通道激活（K_S≠0）时生效（K_S=0 时 law=6 ≡ law=5）
soc_ref_eff = SOC_ref + K_S * e_hat;
lam = lambda + K_soc * (soc_ref_eff - SOC);
if K_S ~= 0
    lam = max(lam, Lambda_Floor);
end
% 可行集 = {0（怠速）} ∪ [0:ECMS_Grid_dP_kW:Gen_P_max]（P_min=0 口径）
N = floor(Gen_P_max / ECMS_Grid_dP_kW) + 1;
Pbest = 0;
Jbest = inf;
nb = numel(bsfc_bp);
for i = 1:N
    Pg = (i - 1) * ECMS_Grid_dP_kW;
    Pbat = P_load - ASSUMED_eta_rect * Pg;
    % SOC 硬约束（优先于 λ）：禁放电 -> 取满足需求的最小可行值
    if SOC <= ECMS_SOC_Discharge_Max
        if Pbat > 1e-9
            continue;
        end
        Pbest = Pg;
        break;
    end
    % SOC 硬约束：禁充电（排除充电网格点）
    if SOC >= ECMS_SOC_Charge_Min && Pbat < 0
        continue;
    end
    % ṁ_f：怠速（Pg=0）用怠速流量，否则 Pg·bsfc(Pg)/3.6e6
    if Pg < 1e-9
        mf = ECMS_Idle_Fuel_kgph / 3600;
    else
        bsfc = bsfc_tbl(1);
        if Pg >= bsfc_bp(nb)
            bsfc = bsfc_tbl(nb);
        elseif Pg > bsfc_bp(1)
            ii = 1;
            while ii < nb - 1 && bsfc_bp(ii + 1) < Pg
                ii = ii + 1;
            end
            w = (Pg - bsfc_bp(ii)) / (bsfc_bp(ii + 1) - bsfc_bp(ii));
            bsfc = bsfc_tbl(ii) + w * (bsfc_tbl(ii + 1) - bsfc_tbl(ii));
        end
        mf = Pg * bsfc / 3.6e6;
    end
    % ṁ_bat,eq：放电正代价，充电负收益（design §3.1 效率链）
    if Pbat > 0
        mbe = Pbat / (ASSUMED_eta_dcdc * ASSUMED_Bat_Eff_Discharge) / 3600;
    else
        mbe = Pbat * (ASSUMED_eta_dcdc * ASSUMED_Bat_Eff_Charge) / 3600;
    end
    J = mf + lam * mbe;
    if J < Jbest
        Jbest = J;
        Pbest = Pg;
    end
end
% 禁放电且需求 > η_rect·P_max（无网格点可满足）-> 尽力最大
if SOC <= ECMS_SOC_Discharge_Max && Pbest < 1e-9 && P_load > ASSUMED_eta_rect * Gen_P_max
    Pbest = Gen_P_max;
end
P = Pbest;
Pheld = Pbest;
end

== matlab function HybridShip_ModelE/05_EMS_Controller/EMS_NN_AECMS/ecms_step ==
  settings: updateMethod=DISCRETE  sampleTime=0.01
  data: t input; P output; P_load input; v_ship input; SOC input; lambda input; K_soc input; SOC_ref input; K_S input; Lambda_Floor input; bsfc_bp input; bsfc_tbl input; W1 input; b1 input; W2 input; b2 input; W3 input; b3 input; XMean input; XStd input; YMean input; YStd input; Ebar input; Escale input; nn_ok input; ASSUMED_eta_rect parameter; ASSUMED_eta_dcdc parameter; ASSUMED_Bat_Eff_Discharge parameter; ASSUMED_Bat_Eff_Charge parameter; Gen_P_max parameter; ECMS_SOC_Discharge_Max parameter; ECMS_SOC_Charge_Min parameter; ECMS_Idle_Fuel_kgph parameter; ECMS_Grid_dP_kW parameter; ECMS_dt_ctrl_s parameter; Pgen_init parameter
function P = ecms_nn(t, P_load, v_ship, SOC, lambda, K_soc, SOC_ref, K_S, Lambda_Floor, bsfc_bp, bsfc_tbl, W1, b1, W2, b2, W3, b3, XMean, XStd, YMean, YStd, Ebar, Escale, nn_ok, ASSUMED_eta_rect, ASSUMED_eta_dcdc, ASSUMED_Bat_Eff_Discharge, ASSUMED_Bat_Eff_Charge, Gen_P_max, ECMS_SOC_Discharge_Max, ECMS_SOC_Charge_Min, ECMS_Idle_Fuel_kgph, ECMS_Grid_dP_kW, ECMS_dt_ctrl_s, Pgen_init)
% NN Predictive A-ECMS（law=7，T-204，design §5，FR-208；2026-08-26 内联恢复）：
%   与 law=6 v2 完全同构：SOC_ref_eff = SOC_ref + K_S·ê_NN；λ_eff = λ₀ + K_soc·(SOC_ref_eff−SOC)；
%   λ_eff = max(λ_eff, Lambda_Floor)（K_S≠0 时生效）。唯一差别是 ê 来源：law=6 从 oracle
%   端口读真值，law=7 由内联 MLP 实时计算（C3/C4 消融唯一差异）。
%   ê_NN = (Ê_NN − Ē_H)/E_scale；Ē_H/E_scale 为与 law=6 相同的 S20 常数。
%   控制周期 ECMS_dt_ctrl_s=1 s：P_load 300 s 环形缓冲 1 s 门控更新；
%   accel = v(t)−v(t−1)（fleet_norm.json feature 口径）；t<lastT 识别新仿真并重置。
%   回退（FR-208）：权重缺失（ECMS_NN_WeightsOK=0）或输入含 NaN -> ê=0（≡law=5 行为）。
persistent lastT Pheld buf k vprev
if isempty(lastT)
    lastT = -1e9;
    Pheld = Pgen_init;
    k = 1;
    buf = zeros(300, 1);
    buf(:) = P_load;
    vprev = v_ship;
end
if t < lastT
    % 新仿真开始：重置缓冲/写指针/速度差基线（与 ecms2.nn_predict_ehat 同语义）
    lastT = t;
    k = 1;
    buf(:) = P_load;
    vprev = v_ship;
end
% 权重/归一化常数经显式输入信号传入（变体内 Constant 引用 workspace 的
% ECMS_NN_*，绕开 R2026a Parameter 端口固化缺陷；见报告 §8 与进展日志）
P = Pheld;
if t - lastT < ECMS_dt_ctrl_s - 1e-9
    return;
end
lastT = t;
if isfinite(P_load)
    buf(k) = P_load;
end
k = mod(k, 300) + 1;
accel = v_ship - vprev;
vprev = v_ship;
ok = nn_ok > 0.5 && isfinite(P_load) && isfinite(v_ship) && isfinite(accel);
% x 构造必须无条件（EMChart 编译器跨块变量缺陷绕过，见报告 §2/§8）；
% 升序重排与 fleet_norm.json feature_layout 一致：xP(1)=P(t-299)...xP(300)=P(t)
xP = [buf(k:300); buf(1:k-1)];
x = [xP; v_ship; accel];
ok = ok && all(isfinite(x));
if ok
xnorm = (x - XMean(:)) ./ XStd(:);
h1 = max(W1.' * xnorm + b1(:), 0);
h2 = max(W2.' * h1 + b2(:), 0);
y_norm = W3.' * h2 + b3;
    Ehat_kWh = y_norm * YStd + YMean;
    e_hat = (Ehat_kWh - Ebar) / Escale;
else
    % 回退：权重缺失或输入非有限 -> ê=0（≡law=5 行为，FR-208）
    e_hat = 0;
end
% 与 law=6 v2 完全一致：自适应 λ（SOC_ref 通道）+ 下限钳位 + 单步网格穷举
soc_ref_eff = SOC_ref + K_S * e_hat;
lam = lambda + K_soc * (soc_ref_eff - SOC);
if K_S ~= 0
    lam = max(lam, Lambda_Floor);
end
N = floor(Gen_P_max / ECMS_Grid_dP_kW) + 1;
Pbest = 0;
Jbest = inf;
nb = numel(bsfc_bp);
for i = 1:N
    Pg = (i - 1) * ECMS_Grid_dP_kW;
    Pbat = P_load - ASSUMED_eta_rect * Pg;
    if SOC <= ECMS_SOC_Discharge_Max
        if Pbat > 1e-9
            continue;
        end
        Pbest = Pg;
        break;
    end
    if SOC >= ECMS_SOC_Charge_Min && Pbat < 0
        continue;
    end
    if Pg < 1e-9
        mf = ECMS_Idle_Fuel_kgph / 3600;
    else
        bsfc = bsfc_tbl(1);
        if Pg >= bsfc_bp(nb)
            bsfc = bsfc_tbl(nb);
        elseif Pg > bsfc_bp(1)
            ii = 1;
            while ii < nb - 1 && bsfc_bp(ii + 1) < Pg
                ii = ii + 1;
            end
            w = (Pg - bsfc_bp(ii)) / (bsfc_bp(ii + 1) - bsfc_bp(ii));
            bsfc = bsfc_tbl(ii) + w * (bsfc_tbl(ii + 1) - bsfc_tbl(ii));
        end
        mf = Pg * bsfc / 3.6e6;
    end
    if Pbat > 0
        mbe = Pbat / (ASSUMED_eta_dcdc * ASSUMED_Bat_Eff_Discharge) / 3600;
    else
        mbe = Pbat * (ASSUMED_eta_dcdc * ASSUMED_Bat_Eff_Charge) / 3600;
    end
    J = mf + lam * mbe;
    if J < Jbest
        Jbest = J;
        Pbest = Pg;
    end
end
if SOC <= ECMS_SOC_Discharge_Max && Pbest < 1e-9 && P_load > ASSUMED_eta_rect * Gen_P_max
    Pbest = Gen_P_max;
end
P = Pbest;
Pheld = Pbest;
end

== matlab function HybridShip_ModelE/06_Genset_System/GensetUnitE_DG1 ==
  settings: updateMethod=DISCRETE  sampleTime=0.01
  data: cmd_start input; P_actual_kW output; cmd_stop input; P_ref_kW input; state output; below_min_flag output; start_count output; DG_P_rated_kW parameter; DG_P_min_kW parameter; DG_ramp_kW_per_s parameter; DG_tau_s parameter; N_ticks_starting parameter; N_ticks_sync parameter; N_ticks_cooldown parameter; Pgen_init parameter
function [P_actual_kW, state, below_min_flag, start_count] = GensetUnitE(...
    cmd_start, cmd_stop, P_ref_kW, ...
    DG_P_rated_kW, DG_P_min_kW, DG_ramp_kW_per_s, DG_tau_s, ...
N_ticks_starting, N_ticks_sync, N_ticks_cooldown, Pgen_init)
%#codegen
% GensetUnitE：单发电机组启停状态机 + 功率链（Model E, FR-418/419, OQ-6 定稿）
%   DG1/DG2 各用一个块实例（同一代码）；固定步 0.01 s，每步调用一次 = 1 tick；
%   状态驻留用整数 tick 计数做转移判据（OQ-6，禁止浮点时间比较）。
%   state: 0=OFF 1=STARTING 2=SYNCHRONIZING 3=ON 4=COOLDOWN（数值状态，供 fuel/log 用）
%   D-4：min up/min down time 不在本 Plant 内（unit commitment 属 B 包 PMS v2）；
%        COOLDOWN 物理驻留 N_ticks_cooldown 表达停机间隔，期间 cmd_start 忽略。
%   aborted-start：STARTING/SYNC 不可中断；cmd_stop 只置 pending_stop，进入 ON 后一拍内执行停机。
%   OFF 态 stop 优先（2026-09-04 主 Agent 裁决）：cmd_start=1 且 cmd_stop=1 时保持 OFF，防停机后无限再启动。
persistent st n_tick pending_stop n_starts P_ramp P_lag
if isempty(st)
    st = 0;                 % 初始 OFF（新状态机初始 OFF；Pgen_init 仅作 P_lag legacy 初值）
    n_tick = 0;             % 当前状态驻留 tick 计数
    pending_stop = false;   % STARTING/SYNC 期间登记的停机请求
    n_starts = 0;           % 完成启动次数（SYNC 完成时 +1，含 aborted-start）
    P_ramp = 0;             % 爬坡状态 [kW]
    P_lag = Pgen_init;      % 一阶惯性状态 [kW]（legacy 常开模型初值兼容语义）
end

P_actual_kW = 0;            % 非 ON 态恒 0；ON 态由功率链覆写
below_min_flag = 0;         % 仅 ON 态置位（ref < P_min；switch 后按最终状态统一判定）

switch st
    case 0 % OFF：cmd_start 触发启动（cmd_stop 有效时 stop 优先，防停机后无限再启动）
        if cmd_start > 0.5 && cmd_stop < 0.5
            st = 1;                  % OFF -> STARTING
            n_tick = 0;
            pending_stop = false;    % n_starts 不在此刻加（SYNC 完成时才计）
            P_ramp = 0;              % 启动从零爬坡
            P_lag = 0;
        end

    case 1 % STARTING：不可中断（aborted-start 只登记）
        n_tick = n_tick + 1;
        if cmd_stop > 0.5
            pending_stop = true;
        end
        if n_tick >= N_ticks_starting
            st = 2;                  % STARTING -> SYNCHRONIZING
            n_tick = 0;
        end

    case 2 % SYNCHRONIZING：不可中断
        n_tick = n_tick + 1;
        if cmd_stop > 0.5
            pending_stop = true;
        end
        if n_tick >= N_ticks_sync
            n_starts = n_starts + 1; % 启动完成（启动燃油由此计量一次）
            st = 3;                  % SYNCHRONIZING -> ON
            n_tick = 0;
        end

    case 3 % ON：功率链 + 停机命令（pending_stop 在此执行）
        if cmd_stop > 0.5 || pending_stop
            pending_stop = false;
            st = 4;                  % ON -> COOLDOWN（断路器分闸，本拍 P=0）
            n_tick = 0;
        else
            % ref clamp [P_min, rated]（below_min_flag 在 switch 后按最终状态统一置位）
            P_ref_c = min(max(P_ref_kW, DG_P_min_kW), DG_P_rated_kW);
            if P_ramp < P_ref_c
                P_ramp = min(P_ramp + DG_ramp_kW_per_s*0.01, P_ref_c);  % 爬坡限幅（0.01 s 步）
            elseif P_ramp > P_ref_c
                P_ramp = max(P_ramp - DG_ramp_kW_per_s*0.01, P_ref_c);
            end
            P_lag = P_lag + (P_ramp - P_lag)*0.01/DG_tau_s;             % 一阶惯性 tau
            P_actual_kW = min(max(P_lag, 0), DG_P_rated_kW);
            % 注：爬坡过渡期 P<P_min 为 registered 过渡（below_min_flag 登记；
            % 燃油侧按 clamp 到 BSFC 下节点(125)查表，见 FuelModelE）
        end

    case 4 % COOLDOWN：P=0；cmd_start 忽略（D-4：物理驻留表达最小停机间隔）
        n_tick = n_tick + 1;
        if n_tick >= N_ticks_cooldown
            st = 0;                  % COOLDOWN -> OFF
            n_tick = 0;
        end

    otherwise % 防御：非法状态归 OFF（无 NaN 路径）
        st = 0;
        n_tick = 0;
end

state = st;                  % 输出为本拍转移后的状态
if st == 3 && P_ref_kW < DG_P_min_kW
    below_min_flag = 1;      % 输出约定：flag=1 当且仅当 state==3 且 ref<P_min（含 ON 入口拍）
end
start_count = n_starts;
end

== matlab function HybridShip_ModelE/06_Genset_System/GensetUnitE_DG2 ==
  settings: updateMethod=DISCRETE  sampleTime=0.01
  data: cmd_start input; P_actual_kW output; cmd_stop input; P_ref_kW input; state output; below_min_flag output; start_count output; DG_P_rated_kW parameter; DG_P_min_kW parameter; DG_ramp_kW_per_s parameter; DG_tau_s parameter; N_ticks_starting parameter; N_ticks_sync parameter; N_ticks_cooldown parameter; Pgen_init parameter
function [P_actual_kW, state, below_min_flag, start_count] = GensetUnitE(...
    cmd_start, cmd_stop, P_ref_kW, ...
    DG_P_rated_kW, DG_P_min_kW, DG_ramp_kW_per_s, DG_tau_s, ...
N_ticks_starting, N_ticks_sync, N_ticks_cooldown, Pgen_init)
%#codegen
% GensetUnitE：单发电机组启停状态机 + 功率链（Model E, FR-418/419, OQ-6 定稿）
%   DG1/DG2 各用一个块实例（同一代码）；固定步 0.01 s，每步调用一次 = 1 tick；
%   状态驻留用整数 tick 计数做转移判据（OQ-6，禁止浮点时间比较）。
%   state: 0=OFF 1=STARTING 2=SYNCHRONIZING 3=ON 4=COOLDOWN（数值状态，供 fuel/log 用）
%   D-4：min up/min down time 不在本 Plant 内（unit commitment 属 B 包 PMS v2）；
%        COOLDOWN 物理驻留 N_ticks_cooldown 表达停机间隔，期间 cmd_start 忽略。
%   aborted-start：STARTING/SYNC 不可中断；cmd_stop 只置 pending_stop，进入 ON 后一拍内执行停机。
%   OFF 态 stop 优先（2026-09-04 主 Agent 裁决）：cmd_start=1 且 cmd_stop=1 时保持 OFF，防停机后无限再启动。
persistent st n_tick pending_stop n_starts P_ramp P_lag
if isempty(st)
    st = 0;                 % 初始 OFF（新状态机初始 OFF；Pgen_init 仅作 P_lag legacy 初值）
    n_tick = 0;             % 当前状态驻留 tick 计数
    pending_stop = false;   % STARTING/SYNC 期间登记的停机请求
    n_starts = 0;           % 完成启动次数（SYNC 完成时 +1，含 aborted-start）
    P_ramp = 0;             % 爬坡状态 [kW]
    P_lag = Pgen_init;      % 一阶惯性状态 [kW]（legacy 常开模型初值兼容语义）
end

P_actual_kW = 0;            % 非 ON 态恒 0；ON 态由功率链覆写
below_min_flag = 0;         % 仅 ON 态置位（ref < P_min；switch 后按最终状态统一判定）

switch st
    case 0 % OFF：cmd_start 触发启动（cmd_stop 有效时 stop 优先，防停机后无限再启动）
        if cmd_start > 0.5 && cmd_stop < 0.5
            st = 1;                  % OFF -> STARTING
            n_tick = 0;
            pending_stop = false;    % n_starts 不在此刻加（SYNC 完成时才计）
            P_ramp = 0;              % 启动从零爬坡
            P_lag = 0;
        end

    case 1 % STARTING：不可中断（aborted-start 只登记）
        n_tick = n_tick + 1;
        if cmd_stop > 0.5
            pending_stop = true;
        end
        if n_tick >= N_ticks_starting
            st = 2;                  % STARTING -> SYNCHRONIZING
            n_tick = 0;
        end

    case 2 % SYNCHRONIZING：不可中断
        n_tick = n_tick + 1;
        if cmd_stop > 0.5
            pending_stop = true;
        end
        if n_tick >= N_ticks_sync
            n_starts = n_starts + 1; % 启动完成（启动燃油由此计量一次）
            st = 3;                  % SYNCHRONIZING -> ON
            n_tick = 0;
        end

    case 3 % ON：功率链 + 停机命令（pending_stop 在此执行）
        if cmd_stop > 0.5 || pending_stop
            pending_stop = false;
            st = 4;                  % ON -> COOLDOWN（断路器分闸，本拍 P=0）
            n_tick = 0;
        else
            % ref clamp [P_min, rated]（below_min_flag 在 switch 后按最终状态统一置位）
            P_ref_c = min(max(P_ref_kW, DG_P_min_kW), DG_P_rated_kW);
            if P_ramp < P_ref_c
                P_ramp = min(P_ramp + DG_ramp_kW_per_s*0.01, P_ref_c);  % 爬坡限幅（0.01 s 步）
            elseif P_ramp > P_ref_c
                P_ramp = max(P_ramp - DG_ramp_kW_per_s*0.01, P_ref_c);
            end
            P_lag = P_lag + (P_ramp - P_lag)*0.01/DG_tau_s;             % 一阶惯性 tau
            P_actual_kW = min(max(P_lag, 0), DG_P_rated_kW);
            % 注：爬坡过渡期 P<P_min 为 registered 过渡（below_min_flag 登记；
            % 燃油侧按 clamp 到 BSFC 下节点(125)查表，见 FuelModelE）
        end

    case 4 % COOLDOWN：P=0；cmd_start 忽略（D-4：物理驻留表达最小停机间隔）
        n_tick = n_tick + 1;
        if n_tick >= N_ticks_cooldown
            st = 0;                  % COOLDOWN -> OFF
            n_tick = 0;
        end

    otherwise % 防御：非法状态归 OFF（无 NaN 路径）
        st = 0;
        n_tick = 0;
end

state = st;                  % 输出为本拍转移后的状态
if st == 3 && P_ref_kW < DG_P_min_kW
    below_min_flag = 1;      % 输出约定：flag=1 当且仅当 state==3 且 ref<P_min（含 ON 入口拍）
end
start_count = n_starts;
end

== matlab function HybridShip_ModelE/07_PMS_v2/PMS_Demand_Policy ==
  settings: updateMethod=DISCRETE  sampleTime=0.01
  data: P_load_gen_kW input; P_gen_req_baseline_kW output; SOC input; N_dispatch_fb input; P_commit_kW output; u_recovery output; P_recovery_actual_kW output; PMS_LoadLPF_tau_s parameter double size=1; PMS_SOC_lo parameter double size=1; PMS_SOC_recovered parameter double size=1; PMS_P_chg_recovery_kW parameter double size=1; DG_P_rated_kW parameter double size=1
function [P_gen_req_baseline_kW, P_commit_kW, u_recovery, P_recovery_actual_kW] = PMSDemandPolicyE(P_load_gen_kW, SOC, N_dispatch_fb, PMS_LoadLPF_tau_s, PMS_SOC_lo, PMS_SOC_recovered, PMS_P_chg_recovery_kW, DG_P_rated_kW)
%#codegen
% PMSDemandPolicyE：Baseline_Demand_Policy 发电需求律（Model E Phase 4-B, FR-432~435, T-002 链 A）
%   依据：.specs/phase4-b-pms-safety/design.md §5.3 + requirements FR-432/433/434/435（AC-417）；
%   brainstorm D-B3（Demand Policy 四数冻结）/ D-B4（P_commit 信号语义方案 b）/ D-B6 / D-B14。
%   角色：07_PMS_v2 内 Baseline source（ems_health_ok=0 时的确定性热备份，D-B7 ③）；
%   advanced EMS source 的 P_gen_req=P_EMS 直送不削减（FR-434），削减只发生在本 Baseline source 内部。
%
%   canonical 功率域（DD-1，genset-side generator-equivalent）：
%     - 全部输入/输出量均为 genset-side generator-equivalent；P_load_gen_kW 已在 07_PMS_v2
%       输入边界经 X_b2g_* 由 bus 侧 ÷ASSUMED_eta_rect 换算入域，本块零换算直用；
%     - PMS_P_chg_recovery_kW=100 kW 为 generator-equivalent recovery bias（≈bus 侧新增发电
%       约 97 kW），禁止表述为"电池 100 kW 实际充电"（DD-1 措辞纪律）。
%
%   输入：P_load_gen_kW 负荷（generator-equivalent）；SOC [-]；N_dispatch_fb dispatch 反馈
%     （在线机组数，**上一拍语义由调用方 UnitDelay 保证**——本函数直接消费当拍入参，
%     内部不再延迟，design §5.3）；PMS_LoadLPF_tau_s / PMS_SOC_lo / PMS_SOC_recovered /
%     PMS_P_chg_recovery_kW 为 FR-435 四参数（全 ENGINEERING_SURROGATE，数值事实源
%     config/ModelE_Control_Parameters.m，敏感性 τ∈{30,120} 冻结登记不扫）；DG_P_rated_kW
%     单机额定（genset 域字面，DD-1）。
%   输出：P_gen_req_baseline_kW = LPF(P_load) + P_recovery_actual（FR-432）；
%     P_commit_kW = LPF(P_load)（commitment 判据信号，不含 recovery 偏置，D-B4 方案 b）；
%     u_recovery SOC 滞回状态（供 logging，design §5.3）；P_recovery_actual_kW 实际恢复偏置。
%
%   离散约定：固定步 0.01 s，每调用一次 = 1 tick；dt=0.01 硬编码于 LPF 更新，
%   若模型固定步长变更须一并重推（同 GensetUnitE OQ-6 口径）。
%   纯 MATLAB：persistent 为唯一状态载体；无 toolbox 依赖；无 evalin/assignin/全局变量。

persistent P_load_filt u_rec
% 注：R2026a MATLAB Function 块解析纪律——persistent 变量不得直接作为输出参量，
% 故滞回状态本体为 u_rec，输出名 u_recovery 在每拍末拷贝输出（语义不变）。
if isempty(P_load_filt)
    P_load_filt = P_load_gen_kW;    % y[0]=x[0]（design §5.3；首拍 LPF 更新数值恒等）
    u_rec = false;                  % FR-433 初值 false
end

% (1) 一阶 LPF 前向欧拉（FR-432）：y[k]=y[k-1]+(Ts/τ)(x[k]-y[k-1])，τ=PMS_LoadLPF_tau_s
%     前向欧拉**非双线性**；标称 τ=60 s 时 Ts/τ≈1.67e-4，远在 0<Ts/τ<2 稳定界内、稳定裕量大
%     （禁称"无条件稳定"，design §5.3 措辞纪律）。
P_load_filt = P_load_filt + (0.01/PMS_LoadLPF_tau_s)*(P_load_gen_kW - P_load_filt);

% (2) SOC 滞回（FR-433，比较符号冻结；D-B3）：<=PMS_SOC_lo 进 / >=PMS_SOC_recovered 出 / 其间保持
if SOC <= PMS_SOC_lo
    u_rec = true;
elseif SOC >= PMS_SOC_recovered
    u_rec = false;
end
u_recovery = u_rec;                 % 输出本拍评估后的滞回状态（供 logging，design §5.3）

% (3) 恢复偏置（FR-434 non-firm/opportunistic）：负荷服务优先，削减只在 Baseline source 内部
%     （recovery 不得单独触发 DG2 启动——commitment 判据用 P_commit_kW，D-B4 结构性规则；
%       EMS 直送不削减，指令/功率 mismatch 经 dispatch 诊断量暴露，D-B6/D-B14）
P_recovery_actual_kW = double(u_rec) * max(0, min(PMS_P_chg_recovery_kW, ...
    DG_P_rated_kW*N_dispatch_fb - P_load_filt));

% (4) 基线发电需求 = LPF(P_load) + 实际恢复偏置（FR-432 / design §5.3）
P_gen_req_baseline_kW = P_load_filt + P_recovery_actual_kW;

% (5) commitment 判据信号 = LPF(P_load)，不含 recovery 偏置（D-B4 方案 b：
%     恢复充电为 opportunistic/non-firm 需求，不得影响启停门槛判定）
P_commit_kW = P_load_filt;
end
